simulink model "sistema2020_4"  (R2020b)
settings: Solver=ode15s  StartTime=0.0  StopTime=10  MaxStep=1E-2  RelTol=1e-3
libraries: fl_lib x10, nesl_utility x6, ee_lib x4, pid_lib x1
settings Model: LastModifiedBy=josue
settings SolverCC: AlgebraicLoopSolver=LineSearch
settings DataIOCC: SaveOutput=off  SignalLogging=off  DSMLogging=off  ReturnWorkspaceOutputs=off  TimeSaveName=t
settings DebuggingCC: AlgebraicLoopMsg=none  ArtificialAlgebraicLoopMsg=none  MaxConsecutiveZCsMsg=none  UnconnectedInputMsg=none  UnconnectedOutputMsg=none  UnconnectedLineMsg=none  ModelReferenceExtraNoncontSigs=none  OperatingPointInterfaceChecksumMismatchMsg=none
settings ModelReferenceCC: UpdateModelReferenceTargets=IfOutOfDate  EnableRefExpFcnMdlSchedulingChecks=off
settings RTWCC: GPUComputeCapability=5.0

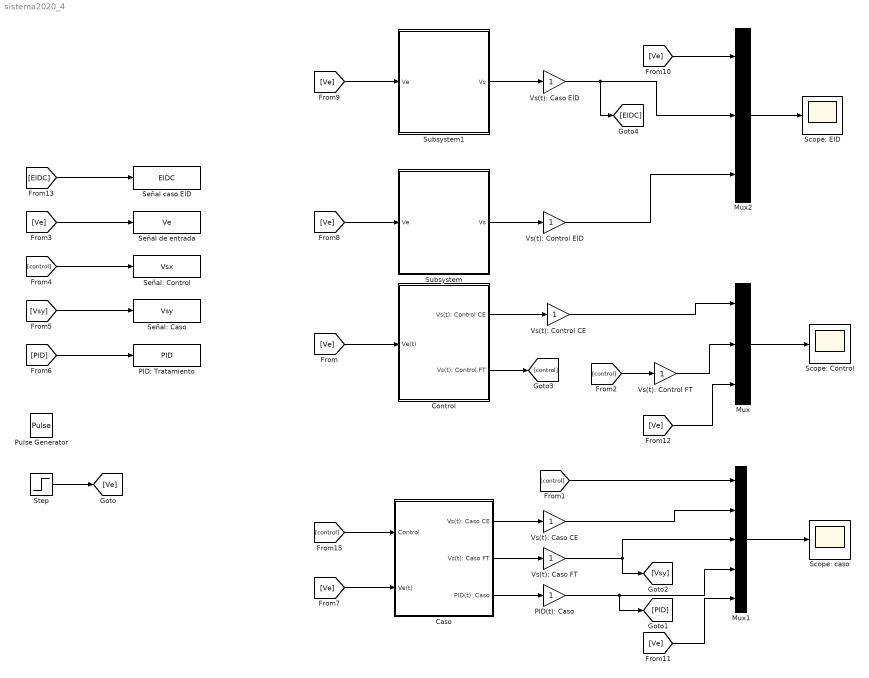
== system sistema2020_4 ==
  Caso : Subsystem
  Control : Subsystem
  Mux : Mux  Inputs=3
  Mux1 : Mux  Inputs=5
  Mux2 : Mux  Inputs=3
  PID(t): Caso : Gain
  PID: Tratamiento : ToWorkspace  VariableName=PID  SampleTime=-1
  Pulse Generator : DiscretePulseGenerator  PulseType=Time based  Period=10  PulseWidth=10  PhaseDelay=1
  Scope: Control : Scope
  Scope: EID : Scope
  Scope: caso : Scope
  Señal caso EID : ToWorkspace  VariableName=EIDC  SampleTime=-1
  Señal de entrada : ToWorkspace  VariableName=Ve  SampleTime=-1
  Señal: Caso : ToWorkspace  VariableName=Vsy  SampleTime=-1
  Señal: Control : ToWorkspace  VariableName=Vsx  SampleTime=-1
  Step : Step  Time=0  Before=1  SampleTime=0
  Subsystem : Subsystem
  Subsystem1 : Subsystem
  Vs(t): Caso CE : Gain
  Vs(t): Caso EID : Gain
  Vs(t): Caso FT : Gain
  Vs(t): Control CE : Gain
  "Vs(t): Control EID " : Gain
  Vs(t): Control FT : Gain
  wires:
  Mux/1 -> Scope: Control/1
  [Ve] -> Control/1(Ve(t))
  Control/1(Vs(t): Control CE) -> Vs(t): Control CE/1
  PID(t): Caso/1 -> [PID], Mux1/4
  Vs(t): Caso CE/1 -> Mux1/2
  Vs(t): Caso FT/1 -> [Vsy], Mux1/3
  Mux1/1 -> Scope: caso/1
  Caso/1(Vs(t): Caso CE) -> Vs(t): Caso CE/1
  Caso/2(Vs(t): Caso FT) -> Vs(t): Caso FT/1
  Caso/3(PID(t): Caso) -> PID(t): Caso/1
  [Ve] -> Caso/2(Ve(t))
  [control] -> Caso/1(Control)
  [control] -> Mux1/1
  [control] -> Vs(t): Control FT/1
  Control/2(Vs(t): Control FT) -> [control]
  [PID] -> PID: Tratamiento/1
  [Vsy] -> Señal: Caso/1
  [control] -> Señal: Control/1
  [Ve] -> Señal de entrada/1
  Step/1 -> [Ve]
  [Ve] -> Subsystem/1(Ve)
  Vs(t): Control CE/1 -> Mux/1
  Subsystem/1(Vs) -> "Vs(t): Control EID "/1
  Vs(t): Control FT/1 -> Mux/2
  [Ve] -> Subsystem1/1(Ve)
  Subsystem1/1(Vs) -> Vs(t): Caso EID/1
  Mux2/1 -> Scope: EID/1
  "Vs(t): Control EID "/1 -> Mux2/3
  Vs(t): Caso EID/1 -> [EIDC], Mux2/2
  [Ve] -> Mux2/1
  [Ve] -> Mux1/5
  [Ve] -> Mux/3
  [EIDC] -> Señal caso EID/1

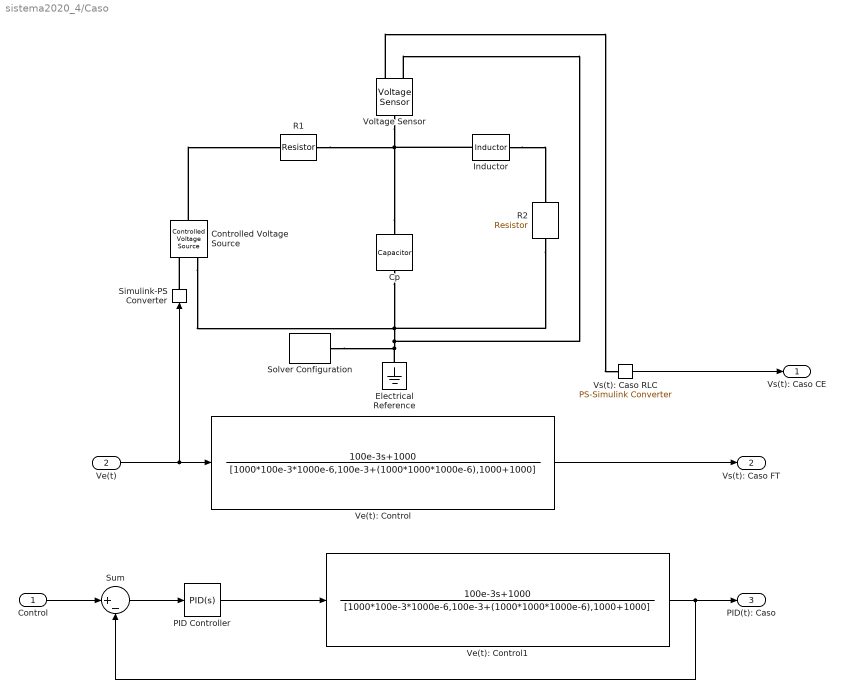
== system sistema2020_4/Caso ==
  Control : Inport
  Ve(t) : Inport  Port=2
  Controlled Voltage Source : fl_lib/Electrical/Electrical Sources/Controlled Voltage Source
  Cp : fl_lib/Electrical/Electrical Elements/Capacitor  c=1000e-6 F  r=1e-6 Ohm  g=0 1/Ohm  i_specify=off  i_priority=None  i=0 A  i_nominal_specify=off  i_nominal_unit=A  i_nominal_value=1  v_specify=off  v_priority=None  v=0 V  v_nominal_specify=off  v_nominal_unit=V  v_nominal_value=1  vc_specify=off  vc_priority=High  vc=0 V  vc_nominal_specify=off  vc_nominal_unit=V  vc_nominal_value=1
  Electrical Reference : fl_lib/Electrical/Electrical Elements/Electrical Reference
  Inductor : fl_lib/Electrical/Electrical Elements/Inductor  l=100e-3 H  r=0 Ohm  g=1e-9 1/Ohm  i_specify=off  i_priority=None  i=0 A  i_nominal_specify=off  i_nominal_unit=A  i_nominal_value=1  v_specify=off  v_priority=None  v=0 V  v_nominal_specify=off  v_nominal_unit=V  v_nominal_value=1  i_L_specify=off  i_L_priority=High  i_L=0 A  i_L_nominal_specify=off  i_L_nominal_unit=A  i_L_nominal_value=1
  PID Controller : pid_lib/PID Controller  Controller=PID  Form=Parallel  TimeDomain=Continuous-time  UseExternalTs=off  SampleTime=-1  IntegratorMethod=Forward Euler  FilterMethod=Forward Euler  ControllerParametersSource=internal  P=1289.29645872171  I=307839.683737193  D=0.179671301047242  UseFilter=on  N=4928.14063077163  TunerSelectOption=Transfer Function Based (PID Tuner App)  InitialConditionSource=internal  InitialConditionForIntegrator=0  InitialConditionForFilter=0  DifferentiatorICPrevScaledInput=0  ExternalReset=none  TrackingMode=off  Kt=1  LimitOutput=off  SatLimitsSource=internal  UpperSaturationLimit=inf  LowerSaturationLimit=-inf  LinearizeAsGain=on  AntiWindupMode=none  Kb=1  POutMin=[]  POutMax=[]  IOutMin=[]  IOutMax=[]  DOutMin=[]  DOutMax=[]  NOutMin=[]  NOutMax=[]  SumOutMin=[]  SumOutMax=[]  SaturationOutMin=[]  SaturationOutMax=[]  PParamMin=[]  PParamMax=[]  IParamMin=[]  IParamMax=[]  DParamMin=[]  DParamMax=[]  NParamMin=[]  NParamMax=[]  KbParamMin=[]  KbParamMax=[]  KtParamMin=[]  KtParamMax=[]  KbOutMin=[]  KbOutMax=[]  KtOutMin=[]  KtOutMax=[]  IntegratorOutMin=[]  IntegratorOutMax=[]  FilterOutMin=[]  FilterOutMax=[]  SumI1OutMin=[]  SumI1OutMax=[]  SumI2OutMin=[]  SumI2OutMax=[]  SumI3OutMin=[]  SumI3OutMax=[]  SumI4OutMin=[]  SumI4OutMax=[]  SumDOutMin=[]  SumDOutMax=[]  DifferentiatorOutMin=[]  DifferentiatorOutMax=[]  FilterDiffOutCoefMin=[]  FilterDiffOutCoefMax=[]  ReciprocalOutMin=[]  ReciprocalOutMax=[]  SumDenOutMin=[]  SumDenOutMax=[]  SumNumOutMin=[]  SumNumOutMax=[]  DivideOutMin=[]  DivideOutMax=[]  UdiffTsProdOutMin=[]  UdiffTsProdOutMax=[]  NTsProdOutMin=[]  NTsProdOutMax=[]  UintegralTsProdOutMin=[]  UintegralTsProdOutMax=[]  UngainTsProdOutMin=[]  UngainTsProdOutMax=[]  IntegratorContinuousStateAttributes=''  IntegratorStateMustResolveToSignalObject=off  IntegratorRTWStateStorageClass=Auto  FilterContinuousStateAttributes=''  FilterStateMustResolveToSignalObject=off  FilterRTWStateStorageClass=Auto  ParallelPVariant=InternalParameters  IdealPVariant=Disabled  IVariant=InternalParameters  DVariant=InternalParameters  IntegratorVariant=Continuous  SatVariant=Disabled  AWVariant=Passthrough  PCopyVariant=Disabled  TRVariant=Disabled  FdbkBlocksVariant=Forward  IdealPFdbkVariant=Disabled  SatFdbkVariant=Disabled  DerivativeFilterVariant=ContFilter  NVariant=InternalParameters  NCopyVariant=Disabled  FilterICVariant=InternalICsFilter  IntegratorICVariant=InternalICs  ExternalResetVariant=Disabled  TRSumVariant=Passthrough  SumFdbkVariant=Disabled  SumVariant=Sum_PID  TsampFilterVariant=InternalTs  TsampNgainVariant=Passthrough  TsampIntegralVariant=Passthrough  ExternalSaturationOutDataTypeStr=Inherit: Same as second input
  R1 : ee_lib/Passive/Resistor  R=1000 Ohm  R_tol=5  enable_R_tol=0  tol_distribution=1  nSigma=4  enable_operating_limits=0  operating_limit_action=2  max_working_voltage=100 V  power_rating=1 W  enable_faults=0  fault_action=1  R_faulted=inf Ohm  enable_temporal_fault=0  t_fault=1 s  enable_behavioral_fault=0  max_permissible_current=1 A  t_fail_on_current=1 s  noise_mode=0  sample_time=1e-3 s  repeatability=1  auto_seed=1196140742  user_seed=0  Tdevice=25 degC  alpha=3.93e-3 1/K  Tmeas=25 degC  thermal_mass=100 J/K  power_derating_T1=70 degC  power_derating_T2=155 degC  operating_temperature_range_vec=[-50, 150] degC  temperature_specify=off  temperature_priority=High  temperature=298.15 K  temperature_nominal_specify=off  temperature_nominal_unit=K  temperature_nominal_value=1
  R2 : ee_lib/Passive/Resistor  R=1000 Ohm  R_tol=5  enable_R_tol=0  tol_distribution=1  nSigma=4  enable_operating_limits=0  operating_limit_action=2  max_working_voltage=100 V  power_rating=1 W  enable_faults=0  fault_action=1  R_faulted=inf Ohm  enable_temporal_fault=0  t_fault=1 s  enable_behavioral_fault=0  max_permissible_current=1 A  t_fail_on_current=1 s  noise_mode=0  sample_time=1e-3 s  repeatability=1  auto_seed=2348838240  user_seed=0  Tdevice=25 degC  alpha=3.93e-3 1/K  Tmeas=25 degC  thermal_mass=100 J/K  power_derating_T1=70 degC  power_derating_T2=155 degC  operating_temperature_range_vec=[-50, 150] degC  temperature_specify=off  temperature_priority=High  temperature=298.15 K  temperature_nominal_specify=off  temperature_nominal_unit=K  temperature_nominal_value=1
  Simulink-PS Converter : nesl_utility/Simulink-PS Converter  PhysicalDomain=network_engine_domain  SubClassName=ps_input  LeftPortType=input  RightPortType=output  PseudoPeriodic=off  Frequencies=[]  NoiseDistribution=none  NoiseParameters=[]  Unit=1  AffineConversion=off  FilteringAndDerivatives=provide  SimscapeFilterOrder=1  InputFilterTimeConstant=0.001  UdotUserProvided=0
  Solver Configuration : nesl_utility/Solver Configuration  PhysicalDomain=network_engine_domain  SubClassName=solver  LeftPortType=input  RightPortType=generic  Tones=[]  Harmonics=[]  SimulateNoise=off  Profile=off  UseLocalSampling=off  EnableSwitchedLinearOptims=on  FrequencyDomain=off  UseCCode=off  RelTol=0.001  AbsTol=1e-06  MinStep=1e-09  ToWorkspace=off  RevertToSquareIcSolve=off  NumHomotopyIterations=100  PhasorMode=off  PhasorModeNumHarmonics=1  DoDC=off  ResidualTolerance=1e-09  UseLocalSolver=off  LocalSolverChoice=NE_BACKWARD_EULER_ADVANCER  LocalSolverSampleTime=0.001  DoFixedCost=off  MaxNonlinIter=3  MaxModeIter=2  ComputeImpulses=off  ImpulseIterations=2  LinearAlgebra=auto  EquationFormulation=NE_TIME_EF  DelaysMemoryBudget=1024  AutomaticFiltering=on  FilteringTimeConstant=0.001  PartitionStorageMethod=AS_NEEDED  PartitionMemoryBudget=1024  PartitionMethod=ROBUST
  Sum : Sum  Inputs=|+-
  Ve(t): Control : TransferFcn  Numerator=[100e-3,1000]  Denominator=[1000*100e-3*1000e-6,100e-3+(1000*1000*1000e-6),1000+1000]
  Ve(t): Control1 : TransferFcn  Numerator=[100e-3,1000]  Denominator=[1000*100e-3*1000e-6,100e-3+(1000*1000*1000e-6),1000+1000]
  Voltage Sensor : fl_lib/Electrical/Electrical Sensors/Voltage Sensor
  "Vs(t): Caso RLC " : nesl_utility/PS-Simulink Converter  PhysicalDomain=network_engine_domain  SubClassName=ps_output  LeftPortType=input  RightPortType=output  PseudoPeriodic=off  Frequencies=[]  Unit=inherit  AffineConversion=off
  Vs(t): Caso CE : Outport
  Vs(t): Caso FT : Outport  Port=2
  PID(t): Caso : Outport  Port=3
  wires:
  Sum/1 -> PID Controller/1
  PID Controller/1 -> Ve(t): Control1/1
  Control/1 -> Sum/1
  Ve(t): Control/1 -> Vs(t): Caso FT/1
  Ve(t): Control1/1 -> Sum/2, PID(t): Caso/1
  "Vs(t): Caso RLC "/1 -> Vs(t): Caso CE/1
  Ve(t)/1 -> Simulink-PS Converter/1, Ve(t): Control/1
  connections:
  Cp/RConn1 -- R2/LConn1 -- Controlled Voltage Source/RConn2 -- Voltage Sensor/RConn2 -- Electrical Reference/LConn1 -- Solver Configuration/RConn1
  Cp/LConn1 -- Voltage Sensor/LConn1 -- R1/LConn1 -- Inductor/LConn1
  Voltage Sensor/RConn1 -- "Vs(t): Caso RLC "/LConn1
  Controlled Voltage Source/LConn1 -- R1/RConn1
  Simulink-PS Converter/RConn1 -- Controlled Voltage Source/RConn1
  Inductor/RConn1 -- R2/RConn1

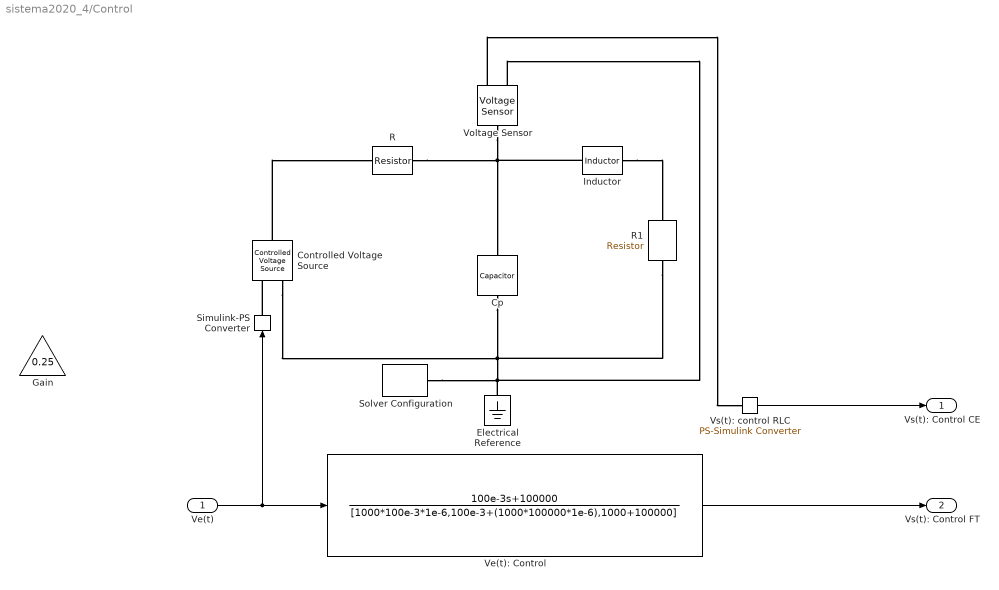
== system sistema2020_4/Control ==
  Ve(t) : Inport
  Controlled Voltage Source : fl_lib/Electrical/Electrical Sources/Controlled Voltage Source
  Cp : fl_lib/Electrical/Electrical Elements/Capacitor  c=1e-6 F  r=1e-6 Ohm  g=0 1/Ohm  i_specify=off  i_priority=None  i=0 A  i_nominal_specify=off  i_nominal_unit=A  i_nominal_value=1  v_specify=off  v_priority=None  v=0 V  v_nominal_specify=off  v_nominal_unit=V  v_nominal_value=1  vc_specify=off  vc_priority=High  vc=0 V  vc_nominal_specify=off  vc_nominal_unit=V  vc_nominal_value=1
  Electrical Reference : fl_lib/Electrical/Electrical Elements/Electrical Reference
  Gain : Gain  Gain=0.25
  Inductor : fl_lib/Electrical/Electrical Elements/Inductor  l=100e-3 H  r=0 Ohm  g=1e-9 1/Ohm  i_specify=off  i_priority=None  i=0 A  i_nominal_specify=off  i_nominal_unit=A  i_nominal_value=1  v_specify=off  v_priority=None  v=0 V  v_nominal_specify=off  v_nominal_unit=V  v_nominal_value=1  i_L_specify=off  i_L_priority=High  i_L=0 A  i_L_nominal_specify=off  i_L_nominal_unit=A  i_L_nominal_value=1
  R : ee_lib/Passive/Resistor  R=1000 Ohm  R_tol=5  enable_R_tol=0  tol_distribution=1  nSigma=4  enable_operating_limits=0  operating_limit_action=2  max_working_voltage=100 V  power_rating=1 W  enable_faults=0  fault_action=1  R_faulted=inf Ohm  enable_temporal_fault=0  t_fault=1 s  enable_behavioral_fault=0  max_permissible_current=1 A  t_fail_on_current=1 s  noise_mode=0  sample_time=1e-3 s  repeatability=1  auto_seed=545404223  user_seed=0  Tdevice=25 degC  alpha=3.93e-3 1/K  Tmeas=25 degC  thermal_mass=100 J/K  power_derating_T1=70 degC  power_derating_T2=155 degC  operating_temperature_range_vec=[-50, 150] degC  temperature_specify=off  temperature_priority=High  temperature=298.15 K  temperature_nominal_specify=off  temperature_nominal_unit=K  temperature_nominal_value=1
  R1 : ee_lib/Passive/Resistor  R=100000 Ohm  R_tol=5  enable_R_tol=0  tol_distribution=1  nSigma=4  enable_operating_limits=0  operating_limit_action=2  max_working_voltage=100 V  power_rating=1 W  enable_faults=0  fault_action=1  R_faulted=inf Ohm  enable_temporal_fault=0  t_fault=1 s  enable_behavioral_fault=0  max_permissible_current=1 A  t_fail_on_current=1 s  noise_mode=0  sample_time=1e-3 s  repeatability=1  auto_seed=3499211588  user_seed=0  Tdevice=25 degC  alpha=3.93e-3 1/K  Tmeas=25 degC  thermal_mass=100 J/K  power_derating_T1=70 degC  power_derating_T2=155 degC  operating_temperature_range_vec=[-50, 150] degC  temperature_specify=off  temperature_priority=High  temperature=298.15 K  temperature_nominal_specify=off  temperature_nominal_unit=K  temperature_nominal_value=1
  Simulink-PS Converter : nesl_utility/Simulink-PS Converter  PhysicalDomain=network_engine_domain  SubClassName=ps_input  LeftPortType=input  RightPortType=output  PseudoPeriodic=off  Frequencies=[]  NoiseDistribution=none  NoiseParameters=[]  Unit=1  AffineConversion=off  FilteringAndDerivatives=provide  SimscapeFilterOrder=1  InputFilterTimeConstant=0.001  UdotUserProvided=0
  Solver Configuration : nesl_utility/Solver Configuration  PhysicalDomain=network_engine_domain  SubClassName=solver  LeftPortType=input  RightPortType=generic  Tones=[]  Harmonics=[]  SimulateNoise=off  Profile=off  UseLocalSampling=off  EnableSwitchedLinearOptims=on  FrequencyDomain=off  UseCCode=off  RelTol=0.001  AbsTol=1e-06  MinStep=1e-09  ToWorkspace=off  RevertToSquareIcSolve=off  NumHomotopyIterations=100  PhasorMode=off  PhasorModeNumHarmonics=1  DoDC=off  ResidualTolerance=1e-09  UseLocalSolver=off  LocalSolverChoice=NE_BACKWARD_EULER_ADVANCER  LocalSolverSampleTime=0.001  DoFixedCost=off  MaxNonlinIter=3  MaxModeIter=2  ComputeImpulses=off  ImpulseIterations=2  LinearAlgebra=auto  EquationFormulation=NE_TIME_EF  DelaysMemoryBudget=1024  AutomaticFiltering=on  FilteringTimeConstant=0.001  PartitionStorageMethod=AS_NEEDED  PartitionMemoryBudget=1024  PartitionMethod=ROBUST
  Ve(t): Control : TransferFcn  Numerator=[100e-3,100000]  Denominator=[1000*100e-3*1e-6,100e-3+(1000*100000*1e-6),1000+100000]
  Voltage Sensor : fl_lib/Electrical/Electrical Sensors/Voltage Sensor
  "Vs(t): control RLC " : nesl_utility/PS-Simulink Converter  PhysicalDomain=network_engine_domain  SubClassName=ps_output  LeftPortType=input  RightPortType=output  PseudoPeriodic=off  Frequencies=[]  Unit=inherit  AffineConversion=off
  Vs(t): Control CE : Outport
  Vs(t): Control FT : Outport  Port=2
  wires:
  "Vs(t): control RLC "/1 -> Vs(t): Control CE/1
  Ve(t): Control/1 -> Vs(t): Control FT/1
  Ve(t)/1 -> Simulink-PS Converter/1, Ve(t): Control/1
  connections:
  Electrical Reference/LConn1 -- Solver Configuration/RConn1 -- Voltage Sensor/RConn2 -- R1/LConn1 -- Controlled Voltage Source/RConn2 -- Cp/RConn1
  Simulink-PS Converter/RConn1 -- Controlled Voltage Source/RConn1
  Controlled Voltage Source/LConn1 -- R/RConn1
  R/LConn1 -- Voltage Sensor/LConn1 -- Inductor/LConn1 -- Cp/LConn1
  Inductor/RConn1 -- R1/RConn1
  Voltage Sensor/RConn1 -- "Vs(t): control RLC "/LConn1

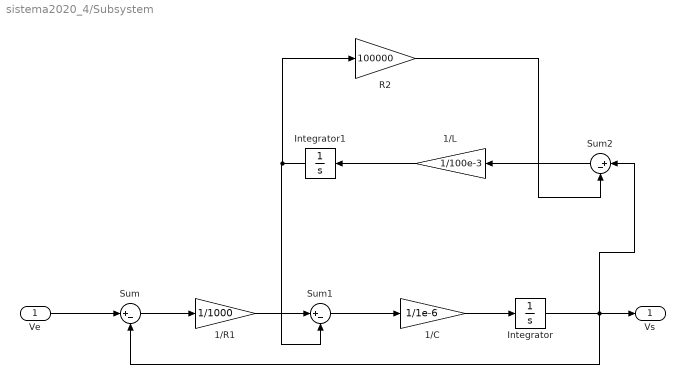
== system sistema2020_4/Subsystem ==
  Ve : Inport
  1/C : Gain  Gain=1/1e-6
  1/L : Gain  Gain=1/100e-3
  1/R1 : Gain  Gain=1/1000
  Integrator : Integrator
  Integrator1 : Integrator
  R2 : Gain  Gain=100000
  Sum : Sum  Inputs=|+-
  Sum1 : Sum  Inputs=|+-
  Sum2 : Sum  Inputs=|+-
  Vs : Outport
  wires:
  Ve/1 -> Sum/1
  Sum/1 -> 1/R1/1
  1/R1/1 -> Sum1/1
  Sum1/1 -> 1/C/1
  1/C/1 -> Integrator/1
  Integrator/1 -> Sum2/1, Sum/2, Vs/1
  1/L/1 -> Integrator1/1
  Integrator1/1 -> R2/1, Sum1/2
  Sum2/1 -> 1/L/1
  R2/1 -> Sum2/2

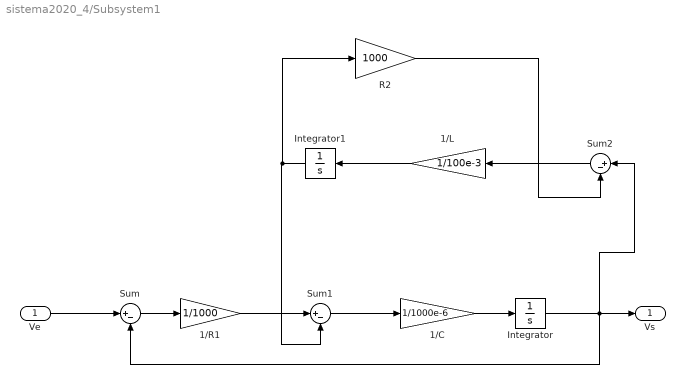
== system sistema2020_4/Subsystem1 ==
  Ve : Inport
  1/C : Gain  Gain=1/1000e-6
  1/L : Gain  Gain=1/100e-3
  1/R1 : Gain  Gain=1/1000
  Integrator : Integrator
  Integrator1 : Integrator
  R2 : Gain  Gain=1000
  Sum : Sum  Inputs=|+-
  Sum1 : Sum  Inputs=|+-
  Sum2 : Sum  Inputs=|+-
  Vs : Outport
  wires:
  Ve/1 -> Sum/1
  Sum/1 -> 1/R1/1
  1/R1/1 -> Sum1/1
  Sum1/1 -> 1/C/1
  1/C/1 -> Integrator/1
  Integrator/1 -> Sum2/1, Sum/2, Vs/1
  1/L/1 -> Integrator1/1
  Integrator1/1 -> R2/1, Sum1/2
  Sum2/1 -> 1/L/1
  R2/1 -> Sum2/2
